simulink model "single_phase_inverter"  (R2026b)
settings: Solver=ode23tb  StopTime=simlength  FixedStep=tc  MaxStep=glb_time.tc
values from neighbouring files (symbols this model uses):
  afe_ctrl = param.afe.ctrl    [init_model.m]
  glb_time = param.glb_time    [init_model.m]
  grid_emu = param.grid.emu    [init_model.m]
  kepsilon = param.spinv.kepsilon    [init_model.m]
  omega_set = param.spinv.omega_set    [init_model.m]
  output_transformer = param.trafo_load.output_transformer    [init_model.m]
  single_phase_inverter_ctrl = param.spinv.ctrl    [init_model.m]
  time_step_ref_1 = param.spinv.ref.time_step_ref_1    [init_model.m]
  time_step_ref_2 = param.spinv.ref.time_step_ref_2    [init_model.m]
  time_step_ref_3 = param.spinv.ref.time_step_ref_3    [init_model.m]
undefined symbols (not defined in the file or in its folder): hwdata
libraries: fl_lib x49, nesl_utility x27, single_phase_transformer_lib x3, phase_shift_filter x2, phase_shift_filter_ccaller x2, lithium_ion_battery x1, three_phase_voltage_emulator x1, power_meter_iec x1, single_phase_transformer x1, three_phase_diode_rectifier x1, three_phase_diode_rectifier_with_thermal_model x1, full_bridge_mosfet_based_with_thermal_model x1
(part 1 of 4)
settings Model: Creator=LTNBDA  LastModifiedBy=d.bagnara
settings SolverCC: AutoInsertRateTranBlk=on  SolverResetMethod=Robust  ZeroCrossAlgorithm=Adaptive  ZeroCrossControl=DisableAll
settings DataIOCC: DSMLogging=off  LimitDataPoints=on  MaxDataPoints=1  ReturnWorkspaceOutputs=off  SaveFormat=Array  SaveOutput=off  SaveTime=off  SignalLogging=off  SignalLoggingSaveFormat=ModelDataLogs
settings OptimizationCC: EfficientMapNaN2IntZero=off  LifeSpan=inf  MemsetInitFltsAndDblsToZero=off
settings DebuggingCC: ArithmeticOperatorsInVariantConditions=warning  FcnCallInpInsideContextMsg=warning  IgnoredZcDiagnostic=none  MergeDetectMultiDrivingBlocksExec=none  MultiTaskCondExecSysMsg=none  MultiTaskDSMMsg=warning  MultiTaskRateTransMsg=warning  SFNoUnconditionalDefaultTransitionDiag=warning  SFUnexpectedBacktrackingDiag=warning  SaveWithParameterizedLinksMsg=none  SignalResolutionControl=TryResolveAllWithWarning  SolverPrmCheckMsg=warning  StateNameClashWarn=warning
settings HardwareCC: ProdEndianess=Unspecified  ProdEqTarget=off  ProdHWDeviceType=Generic->64-bit Embedded Processor (LP64)  ProdIntDivRoundTo=Undefined  ProdLargestAtomicFloat=None  TargetEndianess=LittleEndian  TargetHWDeviceType=MATLAB Host  TargetIntDivRoundTo=Zero  TargetLongLongMode=on
settings ModelReferenceCC: PropagateSignalLabelsOutOfModel=off
settings SFSimCC: CustomCodeUndefinedFunction=UseInterfaceOnly  SimUseLocalCustomCode=off
settings SFSimCC: SimCustomHeaderCode=|
  | #include "phase_shift_flt_simulink.h"
  | #include "sv_pwm.h"
  | #include "rpi.h"
  | #include "rpi_simulink.h"
  | #include "first_harmonic_tracker.h"
  | #include "dqvector_pi.h"
  | #include "dqvector_pi_simulink.h"
  | #include "sv_pwm_simulink.h"
  | #include "dqpll_grid.h"
  | #include "first_harmonic_tracker_simulink.h"
  | #include "dqpll_grid_simulink.h"
  | #include "phase_shift_flt.h"
  | #include "math_f.h"
  | #include "linear_double_integrator_observer_simulink.h"
  | #include "linear_double_integrator_observer.h"
  | #include "sogi_flt_simulink.h"
  | #include "sogi_flt.h"
settings SFSimCC: SimUserIncludeDirs=|
  | include
  | src
settings SFSimCC: SimUserSources=|
  | "rpi.c"
  | "rpi_simulink.c"
  | "dqvector_pi_simulink.c"
  | "dqvector_pi.c"
  | "sv_pwm_simulink.c"
  | "sv_pwm.c"
  | "first_harmonic_tracker_simulink.c"
  | "first_harmonic_tracker.c"
  | "dqpll_grid_simulink.c"
  | "dqpll_grid.c"
  | "phase_shift_flt_simulink.c"
  | "phase_shift_flt.c"
  | "linear_double_integrator_observer_simulink.c"
  | "linear_double_integrator_observer.c"
  | "sogi_flt_simulink.c"
  | "sogi_flt.c"
settings RTWCC: RTWUseLocalCustomCode=off
settings CodeAppCC: StateflowObjectComments=on
settings GRTTargetCC: CombineOutputUpdateFcns=off  GRTInterface=on  TargetLangStandard=C89/C90 (ANSI)
settings ConfigComp: CovExternalEMLEnable=off  CovSaveCumulativeToWorkspaceVar=on  CovSaveSingleToWorkspaceVar=on
settings SimscapeCC: SimscapeNormalizeSystem=off  SimscapeUseEnergyAccounting=off

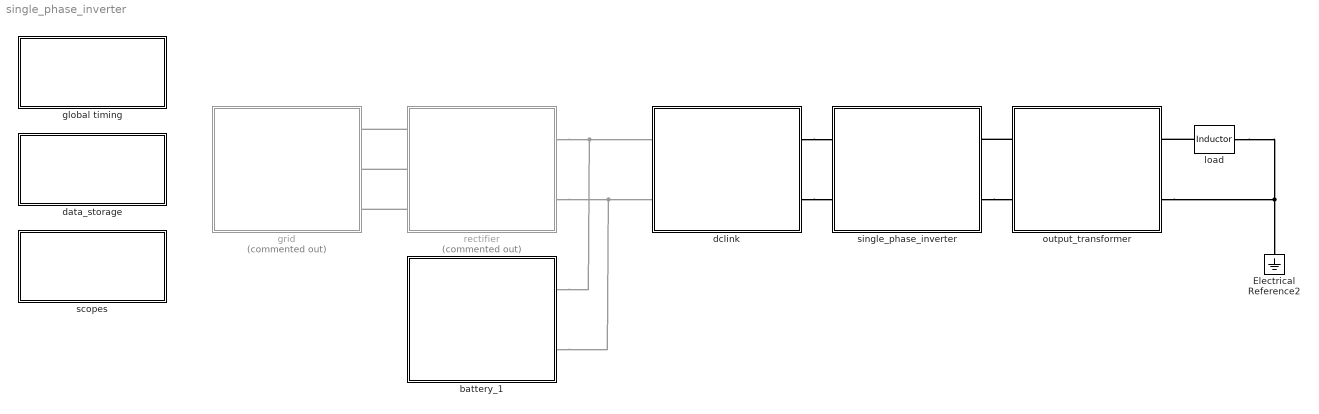
== system single_phase_inverter ==
  Electrical Reference2 : fl_lib/Electrical/Electrical Elements/Electrical Reference
  battery_1 : Subsystem
  data_storage : Subsystem
  dclink : Subsystem
  global timing : Subsystem
  grid : Subsystem  Commented=on
  load : fl_lib/Electrical/Electrical Elements/Inductor  l=lload H  r=rload Ohm  g=1e-9 1/Ohm  i_specify=off  i_priority=None  i=0 A  i_nominal_specify=off  i_nominal_value=1  i_nominal_unit=A  v_specify=off  v_priority=None  v=0 V  v_nominal_specify=off  v_nominal_value=1  v_nominal_unit=V  i_L_specify=off  i_L_priority=High  i_L=0 A  i_L_nominal_specify=off  i_L_nominal_value=1  i_L_nominal_unit=A
  output_transformer : Subsystem
  rectifier : Subsystem  Commented=on
  scopes : Subsystem
  single_phase_inverter : Subsystem
  connections:
  dclink/RConn2 -- single_phase_inverter/LConn2
  dclink/RConn1 -- single_phase_inverter/LConn1
  rectifier/RConn1 -- battery_1/RConn1 -- dclink/LConn1
  rectifier/RConn2 -- battery_1/RConn2 -- dclink/LConn2
  output_transformer/LConn1 -- single_phase_inverter/RConn1
  single_phase_inverter/RConn2 -- output_transformer/LConn2
  output_transformer/RConn2 -- load/RConn1 -- Electrical Reference2/LConn1
  load/LConn1 -- output_transformer/RConn1
  rectifier/LConn3 -- grid/RConn3
  rectifier/LConn2 -- grid/RConn2
  rectifier/LConn1 -- grid/RConn1

== system single_phase_inverter/battery_1 ==
  Electrical Reference : fl_lib/Electrical/Electrical Elements/Electrical Reference
  Inductor : fl_lib/Electrical/Electrical Elements/Inductor  l=1e-3 H  r=0 Ohm  g=1e-9 1/Ohm  i_specify=off  i_priority=None  i=0 A  i_nominal_specify=off  i_nominal_value=1  i_nominal_unit=A  v_specify=off  v_priority=None  v=0 V  v_nominal_specify=off  v_nominal_value=1  v_nominal_unit=V  i_L_specify=off  i_L_priority=High  i_L=0 A  i_L_nominal_specify=off  i_L_nominal_value=1  i_L_nominal_unit=A
  Solver Configuration : nesl_utility/Solver Configuration  PhysicalDomain=network_engine_domain  SubClassName=solver  LeftPortType=input  RightPortType=generic  Tones=[]  Harmonics=[]  SimulateNoise=off  Profile=off  UseLocalSampling=off  EnableSwitchedLinearOptims=on  FrequencyDomain=off  UseCCode=off  RelTol=0.001  AbsTol=0.001  MinStep=1e-09  ToWorkspace=off  RevertToSquareIcSolve=off  NumHomotopyIterations=100  PhasorMode=off  PhasorModeNumHarmonics=1  ConsistencySolver=NEWTON_FTOL  CanonicalOrdering=UNORDERED  OptimizeIntermediates=UNOPTIMIZED  MulticoreSolverChoice=BACKWARD_EULER  IndexReductionMethod=DerivativeReplacement  DoDC=on  ResidualTolerance=1e-3  ConsistencyTolSource=GLOBAL  ConsistencyAbsTol=0.001  ConsistencyRelTol=0.001  ConsistencyTolFactor=0.001  UseLocalSolver=on  LocalSolverChoice=NE_BACKWARD_EULER_ADVANCER  ResolveIndetEquations=on  FunctionEvalNumThread=1  LocalSolverSampleTime=glb_time.tc  DoFixedCost=on  MaxNonlinIter=nonlinear_iterations  MaxModeIter=2  ComputeImpulses=off  ImpulseIterations=2  LinearAlgebra=auto  LinearAlgebraNumThread=0  EquationFormulation=NE_TIME_EF  DelaysMemoryBudget=1024  AutomaticFiltering=on  FilteringTimeConstant=0.001  PartitionStorageMethod=AS_NEEDED  PartitionMemoryBudget=1024  PartitionMethod=BALANCED  MultibodyUseLocalSolver=off  MultibodyLocalSolverChoice=ODE1  MultibodyLocalSolverSampleTime=0.001
  To Workspace14 : ToWorkspace  VariableName=battery_1_data_sim  SampleTime=glb_time.tc
      settings: MaxDataPoints=glb_time.Nc  Decimation=glb_time.decimation_tc
  lithium ion battery : Scope
      settings: ActiveDisplayYMinimum=-808.27997881012811  ActiveDisplayYMaximum=1287.7546757937268  DataLoggingVariableName=ScopeData3
  lithium_ion_battery : lithium_ion_battery/lithium_ion_battery  Q=lithium_ion_battery_1.Q  number_of_cells=lithium_ion_battery_1.number_of_cells  E_1=lithium_ion_battery_1.E_1  E0=lithium_ion_battery_1.E0  E1=lithium_ion_battery_1.E1  E2=lithium_ion_battery_1.E2  E3=lithium_ion_battery_1.E3  Elog=lithium_ion_battery_1.Elog  R0=lithium_ion_battery_1.R0  R1=lithium_ion_battery_1.R1  C1=lithium_ion_battery_1.C1  M=lithium_ion_battery_1.M  alpha=lithium_ion_battery_1.alpha  soc_init=lithium_ion_battery_1.soc_init  ts_battery=glb_time.ts_dab  q1Kalman=lithium_ion_battery_1.q1Kalman  q2Kalman=lithium_ion_battery_1.q2Kalman  q3Kalman=lithium_ion_battery_1.q3Kalman  rKalman=lithium_ion_battery_1.rKalman  tc=glb_time.tc  enable_white_noise_m=0  battery_voltage_init_m=param.battery.nominal_battery_voltage_1
  single_phase_ui_measure : Subsystem
  dc(+) : PMIOPort  Side=Right
  dc(-) : PMIOPort  Port=2  Side=Right
  wires:
  lithium_ion_battery/1 -> To Workspace14/1, lithium ion battery/1
  connections:
  lithium_ion_battery/RConn2 -- single_phase_ui_measure/LConn2 -- Solver Configuration/RConn1 -- Electrical Reference/LConn1
  single_phase_ui_measure/RConn1 -- dc(+)/RConn1
  Inductor/LConn1 -- lithium_ion_battery/RConn1
  dc(-)/RConn1 -- single_phase_ui_measure/RConn2
  single_phase_ui_measure/LConn1 -- Inductor/RConn1

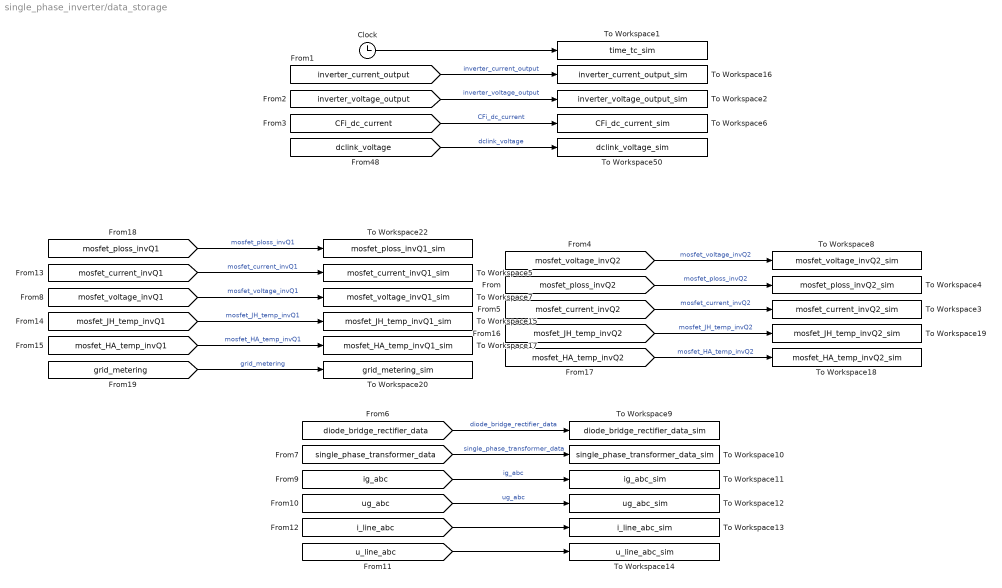
== system single_phase_inverter/data_storage ==
  Clock : Clock
  To Workspace1 : ToWorkspace  VariableName=time_tc_sim  SampleTime=glb_time.tc
      settings: MaxDataPoints=glb_time.Nc  Decimation=glb_time.decimation_tc
  To Workspace10 : ToWorkspace  VariableName=single_phase_transformer_data_sim  SampleTime=glb_time.tc
      settings: MaxDataPoints=glb_time.Nc  Decimation=glb_time.decimation_tc
  To Workspace11 : ToWorkspace  VariableName=ig_abc_sim  SampleTime=glb_time.tc
      settings: MaxDataPoints=glb_time.Nc  Decimation=glb_time.decimation_tc
  To Workspace12 : ToWorkspace  VariableName=ug_abc_sim  SampleTime=glb_time.tc
      settings: MaxDataPoints=glb_time.Nc  Decimation=glb_time.decimation_tc
  To Workspace13 : ToWorkspace  VariableName=i_line_abc_sim  SampleTime=glb_time.tc
      settings: MaxDataPoints=glb_time.Nc  Decimation=glb_time.decimation_tc
  To Workspace14 : ToWorkspace  VariableName=u_line_abc_sim  SampleTime=glb_time.tc
      settings: MaxDataPoints=glb_time.Nc  Decimation=glb_time.decimation_tc
  To Workspace15 : ToWorkspace  VariableName=mosfet_JH_temp_invQ1_sim  SampleTime=glb_time.tc
      settings: MaxDataPoints=glb_time.Nc  Decimation=glb_time.decimation_tc
  To Workspace16 : ToWorkspace  VariableName=inverter_current_output_sim  SampleTime=glb_time.tc
      settings: MaxDataPoints=glb_time.Nc  Decimation=glb_time.decimation_tc
  To Workspace17 : ToWorkspace  VariableName=mosfet_HA_temp_invQ1_sim  SampleTime=glb_time.tc
      settings: MaxDataPoints=glb_time.Nc  Decimation=glb_time.decimation_tc
  To Workspace18 : ToWorkspace  VariableName=mosfet_HA_temp_invQ2_sim  SampleTime=glb_time.tc
      settings: MaxDataPoints=glb_time.Nc  Decimation=glb_time.decimation_tc
  To Workspace19 : ToWorkspace  VariableName=mosfet_JH_temp_invQ2_sim  SampleTime=glb_time.tc
      settings: MaxDataPoints=glb_time.Nc  Decimation=glb_time.decimation_tc
  To Workspace2 : ToWorkspace  VariableName=inverter_voltage_output_sim  SampleTime=glb_time.tc
      settings: MaxDataPoints=glb_time.Nc  Decimation=glb_time.decimation_tc
  To Workspace20 : ToWorkspace  VariableName=grid_metering_sim  SampleTime=glb_time.tc
      settings: MaxDataPoints=glb_time.Nc  Decimation=glb_time.decimation_tc
  To Workspace22 : ToWorkspace  VariableName=mosfet_ploss_invQ1_sim  SampleTime=glb_time.tc
      settings: MaxDataPoints=glb_time.Nc  Decimation=glb_time.decimation_tc
  To Workspace3 : ToWorkspace  VariableName=mosfet_current_invQ2_sim  SampleTime=glb_time.tc
      settings: MaxDataPoints=glb_time.Nc  Decimation=glb_time.decimation_tc
  To Workspace4 : ToWorkspace  VariableName=mosfet_ploss_invQ2_sim  SampleTime=glb_time.tc
      settings: MaxDataPoints=glb_time.Nc  Decimation=glb_time.decimation_tc
  To Workspace5 : ToWorkspace  VariableName=mosfet_current_invQ1_sim  SampleTime=glb_time.tc
      settings: MaxDataPoints=glb_time.Nc  Decimation=glb_time.decimation_tc
  To Workspace50 : ToWorkspace  VariableName=dclink_voltage_sim  SampleTime=glb_time.tc
      settings: MaxDataPoints=glb_time.Nc  Decimation=glb_time.decimation_tc
  To Workspace6 : ToWorkspace  VariableName=CFi_dc_current_sim  SampleTime=glb_time.tc
      settings: MaxDataPoints=glb_time.Nc  Decimation=glb_time.decimation_tc
  To Workspace7 : ToWorkspace  VariableName=mosfet_voltage_invQ1_sim  SampleTime=glb_time.tc
      settings: MaxDataPoints=glb_time.Nc  Decimation=glb_time.decimation_tc
  To Workspace8 : ToWorkspace  VariableName=mosfet_voltage_invQ2_sim  SampleTime=glb_time.tc
      settings: MaxDataPoints=glb_time.Nc  Decimation=glb_time.decimation_tc
  To Workspace9 : ToWorkspace  VariableName=diode_bridge_rectifier_data_sim  SampleTime=glb_time.tc
      settings: MaxDataPoints=glb_time.Nc  Decimation=glb_time.decimation_tc
  wires:
  Clock/1 -> To Workspace1/1
  [inverter_current_output] -> To Workspace16/1  "inverter_current_output"
  [inverter_voltage_output] -> To Workspace2/1  "inverter_voltage_output"
  [CFi_dc_current] -> To Workspace6/1  "CFi_dc_current"
  [mosfet_ploss_invQ1] -> To Workspace22/1  "mosfet_ploss_invQ1"
  [dclink_voltage] -> To Workspace50/1  "dclink_voltage"
  [mosfet_current_invQ1] -> To Workspace5/1  "mosfet_current_invQ1"
  [mosfet_current_invQ2] -> To Workspace3/1  "mosfet_current_invQ2"
  [mosfet_ploss_invQ2] -> To Workspace4/1  "mosfet_ploss_invQ2"
  [mosfet_voltage_invQ1] -> To Workspace7/1  "mosfet_voltage_invQ1"
  [mosfet_voltage_invQ2] -> To Workspace8/1  "mosfet_voltage_invQ2"
  [diode_bridge_rectifier_data] -> To Workspace9/1  "diode_bridge_rectifier_data"
  [single_phase_transformer_data] -> To Workspace10/1  "single_phase_transformer_data"
  [ig_abc] -> To Workspace11/1  "ig_abc"
  [ug_abc] -> To Workspace12/1  "ug_abc"
  [i_line_abc] -> To Workspace13/1
  [u_line_abc] -> To Workspace14/1
  [mosfet_JH_temp_invQ1] -> To Workspace15/1  "mosfet_JH_temp_invQ1"
  [mosfet_HA_temp_invQ1] -> To Workspace17/1  "mosfet_HA_temp_invQ1"
  [mosfet_JH_temp_invQ2] -> To Workspace19/1  "mosfet_JH_temp_invQ2"
  [mosfet_HA_temp_invQ2] -> To Workspace18/1  "mosfet_HA_temp_invQ2"
  [grid_metering] -> To Workspace20/1  "grid_metering"

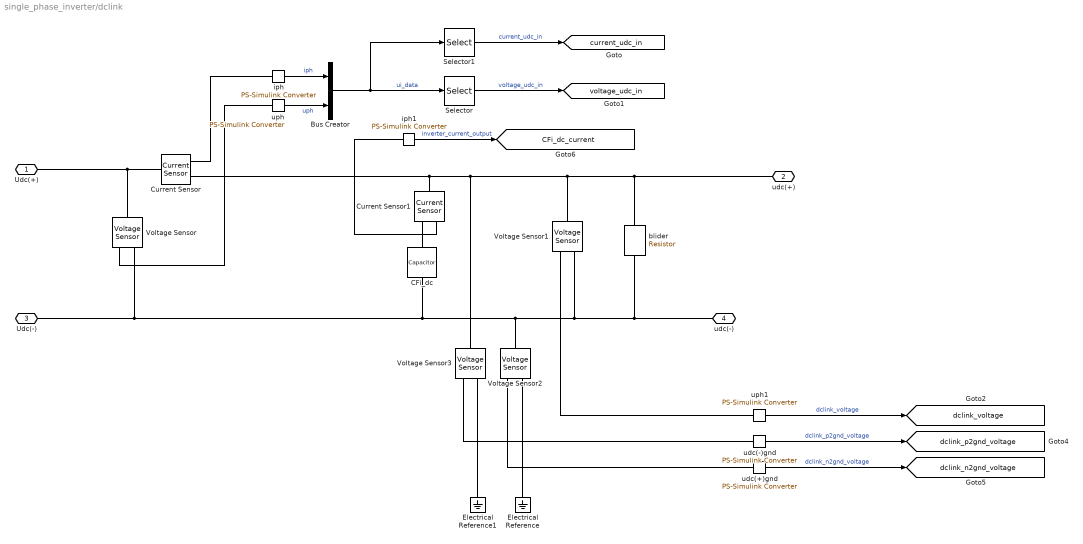
== system single_phase_inverter/dclink ==
  Bus Creator : BusCreator  Inputs=2
  CFi_dc : fl_lib/Electrical/Electrical Elements/Capacitor  c=hwdata.single_phase_inverter.CFi F  r=hwdata.single_phase_inverter.RCFi Ohm  g=0 1/Ohm  i_specify=off  i_priority=None  i=0 A  i_nominal_specify=off  i_nominal_value=1  i_nominal_unit=A  v_specify=off  v_priority=None  v=0 V  v_nominal_specify=off  v_nominal_value=1  v_nominal_unit=V  vc_specify=off  vc_priority=High  vc=0 V  vc_nominal_specify=off  vc_nominal_value=1  vc_nominal_unit=V
  Current Sensor : fl_lib/Electrical/Electrical Sensors/Current Sensor
  Current Sensor1 : fl_lib/Electrical/Electrical Sensors/Current Sensor
  Electrical Reference : fl_lib/Electrical/Electrical Elements/Electrical Reference
  Electrical Reference1 : fl_lib/Electrical/Electrical Elements/Electrical Reference
  Selector : Selector  InputPortWidth=2  IndexOptions=Index vector (dialog)  Indices=2  OutputSizes=1  RuntimeRangeChecks=off
  Selector1 : Selector  InputPortWidth=2  IndexOptions=Index vector (dialog)  Indices=1  OutputSizes=1  RuntimeRangeChecks=off
  Voltage Sensor{,1..3} (4 alike) : fl_lib/Electrical/Electrical Sensors/Voltage Sensor
  blider : fl_lib/Electrical/Electrical Elements/Resistor  R=1200 Ohm  i_specify=off  i_priority=None  i=0 A  i_nominal_specify=off  i_nominal_value=1  i_nominal_unit=A  v_specify=off  v_priority=None  v=0 V  v_nominal_specify=off  v_nominal_value=1  v_nominal_unit=V
  iph : nesl_utility/PS-Simulink Converter  PhysicalDomain=network_engine_domain  SubClassName=ps_output  LeftPortType=input  RightPortType=output  PseudoPeriodic=off  Frequencies=[]  VectorFormat=1-D array  Unit=A  AffineConversion=off
  iph1 : nesl_utility/PS-Simulink Converter  PhysicalDomain=network_engine_domain  SubClassName=ps_output  LeftPortType=input  RightPortType=output  PseudoPeriodic=off  Frequencies=[]  VectorFormat=1-D array  Unit=A  AffineConversion=off
  udc(+)gnd : nesl_utility/PS-Simulink Converter  PhysicalDomain=network_engine_domain  SubClassName=ps_output  LeftPortType=input  RightPortType=output  PseudoPeriodic=off  Frequencies=[]  VectorFormat=1-D array  Unit=V  AffineConversion=off
  udc(-)gnd : nesl_utility/PS-Simulink Converter  PhysicalDomain=network_engine_domain  SubClassName=ps_output  LeftPortType=input  RightPortType=output  PseudoPeriodic=off  Frequencies=[]  VectorFormat=1-D array  Unit=V  AffineConversion=off
  uph : nesl_utility/PS-Simulink Converter  PhysicalDomain=network_engine_domain  SubClassName=ps_output  LeftPortType=input  RightPortType=output  PseudoPeriodic=off  Frequencies=[]  VectorFormat=1-D array  Unit=V  AffineConversion=off
  uph1 : nesl_utility/PS-Simulink Converter  PhysicalDomain=network_engine_domain  SubClassName=ps_output  LeftPortType=input  RightPortType=output  PseudoPeriodic=off  Frequencies=[]  VectorFormat=1-D array  Unit=V  AffineConversion=off
  Udc(+) : PMIOPort  Side=Left
  udc(+) : PMIOPort  Port=2  Side=Right
  Udc(-) : PMIOPort  Port=3  Side=Left
  udc(-) : PMIOPort  Port=4  Side=Right
  tag scope: CFi_dc_current=global, current_udc_in=global, dclink_n2gnd_voltage=global, dclink_p2gnd_voltage=global, dclink_voltage=global, voltage_udc_in=global
  wires:
  Bus Creator/1 -> Selector/1, Selector1/1  "ui_data"
  iph/1 -> Bus Creator/1  "iph"
  uph/1 -> Bus Creator/2  "uph"
  Selector1/1 -> [current_udc_in]  "current_udc_in"
  Selector/1 -> [voltage_udc_in]  "voltage_udc_in"
  iph1/1 -> [CFi_dc_current]  "inverter_current_output"
  udc(+)gnd/1 -> [dclink_n2gnd_voltage]  "dclink_n2gnd_voltage"
  uph1/1 -> [dclink_voltage]  "dclink_voltage"
  udc(-)gnd/1 -> [dclink_p2gnd_voltage]  "dclink_p2gnd_voltage"
  connections:
  iph/LConn1 -- Current Sensor/RConn1
  Voltage Sensor/LConn1 -- Current Sensor/LConn1 -- Udc(+)/RConn1
  Voltage Sensor/RConn1 -- uph/LConn1
  CFi_dc/RConn1 -- Voltage Sensor1/RConn2 -- udc(-)/RConn1 -- blider/RConn1 -- Voltage Sensor2/LConn1 -- Voltage Sensor/RConn2 -- Udc(-)/RConn1
  udc(+)/RConn1 -- blider/LConn1 -- Voltage Sensor1/LConn1 -- Voltage Sensor3/LConn1 -- Current Sensor/RConn2 -- Current Sensor1/LConn1
  Current Sensor1/RConn2 -- CFi_dc/LConn1
  Electrical Reference1/LConn1 -- Voltage Sensor3/RConn2
  udc(-)gnd/LConn1 -- Voltage Sensor3/RConn1
  Voltage Sensor2/RConn1 -- udc(+)gnd/LConn1
  Electrical Reference/LConn1 -- Voltage Sensor2/RConn2
  Voltage Sensor1/RConn1 -- uph1/LConn1
  Current Sensor1/RConn1 -- iph1/LConn1

== system single_phase_inverter/global timing ==
  Unit Delay : UnitDelay  SampleTime=glb_time.tc
  time_afe1 : Subsystem  mask{k=1}
      mask prompts: k "Time Gain"
      mask Display:
      | disp('time-gen');
      | port_label('input', 1, 'crt');
      | port_label('output', 1, 'tout');
  time_afe3 : Subsystem  mask{k=1}
      mask prompts: k "Time Gain"
      mask Display:
      | disp('time-gen');
      | port_label('output', 1, 'tout');
  tag scope: master_time=global, time_inv_module_1=global
  wires:
  time_afe1/1(Out1) -> [time_inv_module_1]
  time_afe3/1(Out1) -> [master_time]
  [local_time_corr_llc_mod1] -> Unit Delay/1
  Unit Delay/1 -> time_afe1/1(correction_time)

== system single_phase_inverter/grid ==
  grid_emulator : Subsystem
  power meter iec : power_meter_iec/power meter iec  period=10e-3  ts=glb_time.tc  enable_time=0.025
  threephase_vi_measures : Subsystem
  ua : PMIOPort  Side=Right
  ub : PMIOPort  Port=2  Side=Right
  uc : PMIOPort  Port=3  Side=Right
  tag scope: grid_metering=global
  wires:
  [ug_abc] -> power meter iec/2
  [grid_pulsation_emulator] -> power meter iec/4
  [ig_abc] -> power meter iec/3
  [grid_phase_emulator] -> power meter iec/1
  power meter iec/1 -> [grid_metering]
  connections:
  threephase_vi_measures/LConn3 -- grid_emulator/RConn3
  threephase_vi_measures/LConn1 -- grid_emulator/RConn1
  threephase_vi_measures/RConn2 -- ub/RConn1
  threephase_vi_measures/LConn2 -- grid_emulator/RConn2
  threephase_vi_measures/RConn1 -- ua/RConn1
  threephase_vi_measures/RConn3 -- uc/RConn1

== system single_phase_inverter/output_transformer ==
  single_phase_transformer : single_phase_transformer/single_phase_transformer  lm_trafo=output_transformer.Lm1  m1=output_transformer.n1  m2=output_transformer.n2  rd1_trafo=output_transformer.Rd1  rd2_trafo=0  ld1_trafo=2*output_transformer.Ld1  ld2_trafo=0  rfe_trafo=output_transformer.Rfe1  length_core=1  mu0=1.256637e-6  mur=1200
  single_phase_transformer - scope : Scope
      settings: ActiveDisplayYMinimum=-52667.127888169394  ActiveDisplayYMaximum=52594.361496045676  DataLoggingVariableName=ScopeData11
  u1(+) : PMIOPort  Side=Left
  u2(+) : PMIOPort  Port=2  Side=Right
  u1(-) : PMIOPort  Port=3  Side=Left
  u2(-) : PMIOPort  Port=4  Side=Right
  tag scope: single_phase_transformer_data=global
  wires:
  single_phase_transformer/1 -> [single_phase_transformer_data], single_phase_transformer - scope/1
  connections:
  single_phase_transformer/LConn2 -- u1(-)/RConn1
  single_phase_transformer/LConn1 -- u1(+)/RConn1
  single_phase_transformer/RConn1 -- u2(+)/RConn1
  single_phase_transformer/RConn2 -- u2(-)/RConn1

== system single_phase_inverter/rectifier ==
  H5_filter : Subsystem  Commented=on
  H7_filter : Subsystem  Commented=on
  three phase diode rectifier : three_phase_diode_rectifier/three phase diode rectifier  Commented=on  Vf_diode_rectifier=diode.rectifier.Vf  Rdon_diode_rectifier=diode.rectifier.Rdon  Csnubber=igbt.inv.Csnubber  Rsnubber=igbt.inv.Rsnubber
  three_phase_diode_rectifier_with_thermal_model : three_phase_diode_rectifier_with_thermal_model/three_phase_diode_rectifier_with_thermal_model  Vf_diode_rectifier=diode.rectifier.Vf  Rdon_diode_rectifier=diode.rectifier.Rdon  mass_heatsink_m=heatsink.no_weight  specific_heat_m=heatsink.cp  rth_diode_JH_m=igbt.inv.Rth_diode_JH  rth_diode_HA_m=Rth_mosfet_HA  Csnubber=igbt.inv.Csnubber  Rsnubber=igbt.inv.Rsnubber
      link override diode_3/Goto2: GotoTag=diode3_JH_temperature
  us_a : PMIOPort  Side=Left
  us_b : PMIOPort  Port=2  Side=Left
  us_c : PMIOPort  Port=3  Side=Left
  Udc(+) : PMIOPort  Port=4  Side=Right
  Udc(-) : PMIOPort  Port=5  Side=Right
  tag scope: diode_bridge_rectifier_data=global
  wires:
  three_phase_diode_rectifier_with_thermal_model/1 -> [diode_bridge_rectifier_data]
  connections:
  Udc(+)/RConn1 -- three_phase_diode_rectifier_with_thermal_model/RConn1 -- three phase diode rectifier/RConn1
  Udc(-)/RConn1 -- three_phase_diode_rectifier_with_thermal_model/RConn2 -- three phase diode rectifier/RConn2
  H5_filter/LConn1 -- us_a/RConn1 -- three_phase_diode_rectifier_with_thermal_model/LConn1 -- three phase diode rectifier/LConn1 -- H7_filter/LConn1
  H5_filter/LConn2 -- us_b/RConn1 -- three phase diode rectifier/LConn2 -- three_phase_diode_rectifier_with_thermal_model/LConn2 -- H7_filter/LConn2
  H5_filter/LConn3 -- us_c/RConn1 -- three_phase_diode_rectifier_with_thermal_model/LConn3 -- three phase diode rectifier/LConn3 -- H7_filter/LConn3

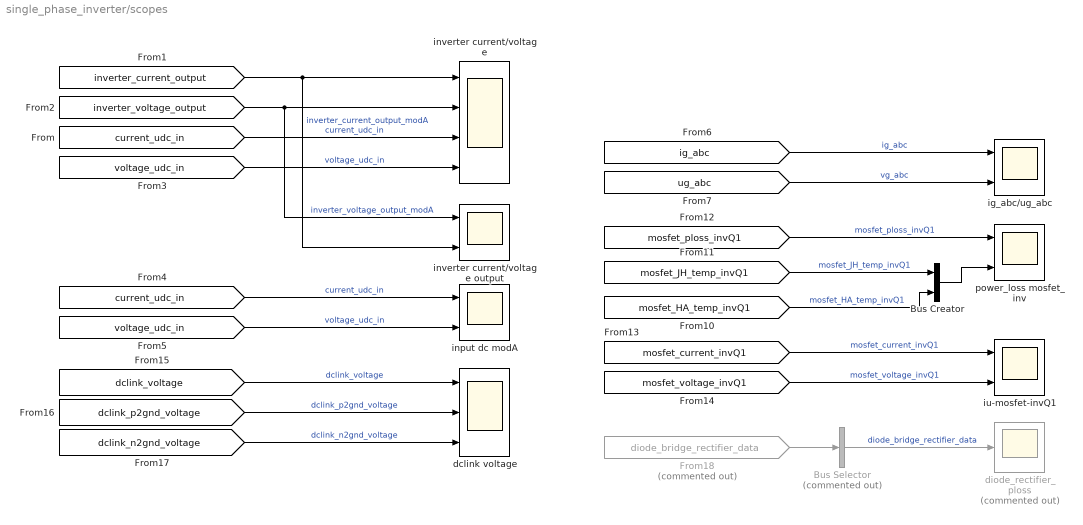
== system single_phase_inverter/scopes ==
  Bus Creator : BusCreator  Inputs=2
  Bus Selector : BusSelector  Commented=on  OutputSignals=diode1_ploss,diode6_ploss,diode5_ploss,diode4_ploss,diode3_ploss,diode2_ploss  OutputAsBus=on
  From18 : From  Commented=on  GotoTag=diode_bridge_rectifier_data
  dclink voltage : Scope  NumInputPorts=3
      settings: SampleTime=glb_time.tc  ActiveDisplayString=3  ActiveDisplayYMinimum=-458.99159991109462  ActiveDisplayYMaximum=51.251012962530893  DataLoggingVariableName=ScopeData9
  diode_rectifier_ploss : Scope  Commented=on
      settings: ActiveDisplayYMinimum=-388.41488046396341  ActiveDisplayYMaximum=3494.091610714474  DataLoggingVariableName=ScopeData13
  ig_abc/ug_abc : Scope  NumInputPorts=2
      settings: SampleTime=glb_time.tc  ActiveDisplayYMinimum=-432.03154642527051  ActiveDisplayYMaximum=443.5760585618213  DataLoggingVariableName=ScopeData5
  input dc modA : Scope  NumInputPorts=2
      settings: SampleTime=glb_time.tc  ActiveDisplayYMinimum=-178.52925477225054  ActiveDisplayYMaximum=1606.7629734926184  DataLoggingVariableName=ScopeData4
  inverter current/voltage : Scope  NumInputPorts=4
      settings: ActiveDisplayString=3  ActiveDisplayYMinimum=-178.52926094214885  ActiveDisplayYMaximum=1606.7629741781627
  inverter current/voltage output : Scope  NumInputPorts=2
      settings: ActiveDisplayYMinimum=-156.50578790248869  ActiveDisplayYMaximum=540.48726644352541
  iu-mosfet-invQ1 : Scope  NumInputPorts=2
      settings: SampleTime=glb_time.tc  ActiveDisplayYMinimum=-1884.5917198054758  ActiveDisplayYMaximum=2532.7760155502147  DataLoggingVariableName=ScopeData7
  power_loss mosfet_inv : Scope  NumInputPorts=2
      settings: SampleTime=glb_time.tc  ActiveDisplayYMinimum=-70.3597503046535  ActiveDisplayYMaximum=633.23512274412  DataLoggingVariableName=ScopeData6
  wires:
  [current_udc_in] -> inverter current/voltage/3  "current_udc_in"
  [inverter_voltage_output] -> inverter current/voltage/2, inverter current/voltage output/1  "inverter_voltage_output_modA"
  [inverter_current_output] -> inverter current/voltage/1, inverter current/voltage output/2  "inverter_current_output_modA"
  [voltage_udc_in] -> inverter current/voltage/4  "voltage_udc_in"
  [current_udc_in] -> input dc modA/1  "current_udc_in"
  [voltage_udc_in] -> input dc modA/2  "voltage_udc_in"
  [ug_abc] -> ig_abc/ug_abc/2  "vg_abc"
  [ig_abc] -> ig_abc/ug_abc/1  "ig_abc"
  [mosfet_ploss_invQ1] -> power_loss mosfet_inv/1  "mosfet_ploss_invQ1"
  [mosfet_JH_temp_invQ1] -> Bus Creator/1  "mosfet_JH_temp_invQ1"
  [mosfet_HA_temp_invQ1] -> Bus Creator/2  "mosfet_HA_temp_invQ1"
  Bus Creator/1 -> power_loss mosfet_inv/2
  [mosfet_current_invQ1] -> iu-mosfet-invQ1/1  "mosfet_current_invQ1"
  [mosfet_voltage_invQ1] -> iu-mosfet-invQ1/2  "mosfet_voltage_invQ1"
  [dclink_voltage] -> dclink voltage/1  "dclink_voltage"
  [dclink_p2gnd_voltage] -> dclink voltage/2  "dclink_p2gnd_voltage"
  [dclink_n2gnd_voltage] -> dclink voltage/3  "dclink_n2gnd_voltage"
  From18/1 -> Bus Selector/1
  Bus Selector/1 -> diode_rectifier_ploss/1  "diode_bridge_rectifier_data"

== system single_phase_inverter/single_phase_inverter ==
  Current Sensor : fl_lib/Electrical/Electrical Sensors/Current Sensor
  Voltage Sensor1 : fl_lib/Electrical/Electrical Sensors/Voltage Sensor
  iph : nesl_utility/PS-Simulink Converter  PhysicalDomain=network_engine_domain  SubClassName=ps_output  LeftPortType=input  RightPortType=output  PseudoPeriodic=off  Frequencies=[]  VectorFormat=1-D array  Unit=A  AffineConversion=off
  single phase inverter : Subsystem
      settings: PortSchema="{\"entries\":[{\"content\":{\"sides\":[{\"content\":{\"connectorIds\":[\"LConn1\",\"LConn2\"]},\"type\":\"ConnectorPlacement.EquallySpacedRectSide\",\"uuid\":\"4fcf4fea-d38f-431b-8a91-be3ce9782faf\"},{\"content\":{\"connectorIds\":[\"RConn1\",\"RConn2\"],\"side\":\"RIGHT\"},\"type\":\"ConnectorPlacement.EquallySpacedRectSide\",\"uuid\":\"0aa56277-92e9-4e3b-84c7-43398254a4d8\"},{\"content\":{\"connectorIds\":[\"In1\"],\"side\":\"TOP\"},\"type\":\"ConnectorPlacement.EquallySpacedRectSide\",\"uuid\":\"5cd150dc-bcaf-4cd7-b2a8-3db203726730\"}]},\"type\":\"ConnectorPlacement.EquallySpacedConnector\",\"uuid\":\"bf8194c4-c327-4d40-bea4-f1e7617f80b4\"}],\"packageUris\":[\"http://schema.mathworks.com/mf0/Connector/R2020b\"],\"version\":\"1.0\"}"
  single phase inverter control : Subsystem
  uph1 : nesl_utility/PS-Simulink Converter  PhysicalDomain=network_engine_domain  SubClassName=ps_output  LeftPortType=input  RightPortType=output  PseudoPeriodic=off  Frequencies=[]  VectorFormat=1-D array  Unit=V  AffineConversion=off
  uac(+) : PMIOPort  Side=Right
  uac(-) : PMIOPort  Port=2  Side=Right
  udc(+) : PMIOPort  Port=3  Side=Left
  udc(-) : PMIOPort  Port=4  Side=Left
  tag scope: inverter_current_output=global, inverter_voltage_output=global
  wires:
  single phase inverter control/1(gate_cmds) -> single phase inverter/1(gate_commands)
  iph/1 -> [inverter_current_output]  "inverter_current_output"
  uph1/1 -> [inverter_voltage_output]  "inverter_voltage_output"
  connections:
  Current Sensor/LConn1 -- single phase inverter/LConn1
  uac(-)/RConn1 -- single phase inverter/LConn2 -- Voltage Sensor1/RConn2
  Voltage Sensor1/RConn1 -- uph1/LConn1
  iph/LConn1 -- Current Sensor/RConn1
  uac(+)/RConn1 -- Current Sensor/RConn2 -- Voltage Sensor1/LConn1
  udc(+)/RConn1 -- single phase inverter/RConn1
  udc(-)/RConn1 -- single phase inverter/RConn2

== system single_phase_inverter/battery_1/single_phase_ui_measure ==
  Bus Creator : BusCreator  Inputs=2
  Current Sensor : fl_lib/Electrical/Electrical Sensors/Current Sensor
  Selector : Selector  InputPortWidth=2  IndexOptions=Index vector (dialog)  Indices=2  OutputSizes=1  RuntimeRangeChecks=off
  Selector1 : Selector  InputPortWidth=2  IndexOptions=Index vector (dialog)  Indices=1  OutputSizes=1  RuntimeRangeChecks=off
  Terminator : Terminator
  Terminator1 : Terminator
  Voltage Sensor : fl_lib/Electrical/Electrical Sensors/Voltage Sensor
  dab input modA : Scope  NumInputPorts=2
      settings: SampleTime=glb_time.tc  ActiveDisplayYMinimum=1239.6508899029441  ActiveDisplayYMaximum=1249.6536701415532  DataLoggingVariableName=ScopeData2
  iph : nesl_utility/PS-Simulink Converter  PhysicalDomain=network_engine_domain  SubClassName=ps_output  LeftPortType=input  RightPortType=output  PseudoPeriodic=off  Frequencies=[]  VectorFormat=1-D array  Unit=A  AffineConversion=off
  uph : nesl_utility/PS-Simulink Converter  PhysicalDomain=network_engine_domain  SubClassName=ps_output  LeftPortType=input  RightPortType=output  PseudoPeriodic=off  Frequencies=[]  VectorFormat=1-D array  Unit=V  AffineConversion=off
  Udc(+) : PMIOPort  Side=Left
  udc(+) : PMIOPort  Port=2  Side=Right
  Udc(-) : PMIOPort  Port=3  Side=Left
  udc(-) : PMIOPort  Port=4  Side=Right
  tag scope: current_battery_1=global, voltage_battery_1=global
  wires:
  Bus Creator/1 -> Selector/1, Selector1/1  "ui_data"
  iph/1 -> Bus Creator/1  "iph"
  uph/1 -> Bus Creator/2  "uph"
  Selector1/1 -> [current_battery_1], dab input modA/1  "current_battery"
  Selector/1 -> dab input modA/2, [voltage_battery_1]  "voltage_battery"
  [current_battery_1] -> Terminator/1
  [voltage_battery_1] -> Terminator1/1
  connections:
  iph/LConn1 -- Current Sensor/RConn1
  Voltage Sensor/LConn1 -- Current Sensor/LConn1 -- Udc(+)/RConn1
  Current Sensor/RConn2 -- udc(+)/RConn1
  Voltage Sensor/RConn1 -- uph/LConn1
  Voltage Sensor/RConn2 -- Udc(-)/RConn1 -- udc(-)/RConn1

== system single_phase_inverter/global timing/time_afe1 ==
  correction_time : Inport
  Constant : Constant
  Gain : Gain  Gain=k
  Product : Product
  Sum : Sum  Inputs=|++
  time_1 : Clock
  Out1 : Outport
  wires:
  time_1/1 -> Gain/1
  Gain/1 -> Product/1
  Product/1 -> Out1/1
  correction_time/1 -> Sum/1
  Sum/1 -> Product/2
  Constant/1 -> Sum/2

== system single_phase_inverter/global timing/time_afe3 ==
  Gain : Gain  Gain=k
  time_1 : Clock
  Out1 : Outport
  wires:
  Gain/1 -> Out1/1
  time_1/1 -> Gain/1

== system single_phase_inverter/grid/grid_emulator ==
  3ph_Dyg : Subsystem
  Bus Selector : BusSelector  OutputSignals=ua_grid_emu,ub_grid_emu,uc_grid_emu
  Bus Selector1 : BusSelector  OutputSignals=gamma_grid_emulator,omega_grid_emulator
  Controlled Voltage Source : fl_lib/Electrical/Electrical Sources/Controlled Voltage Source
  Controlled Voltage Source1 : fl_lib/Electrical/Electrical Sources/Controlled Voltage Source
  Controlled Voltage Source2 : fl_lib/Electrical/Electrical Sources/Controlled Voltage Source
  Electrical Reference : fl_lib/Electrical/Electrical Elements/Electrical Reference
  Simulink-PS Converter : nesl_utility/Simulink-PS Converter  PhysicalDomain=network_engine_domain  SubClassName=ps_input  LeftPortType=input  RightPortType=output  PseudoPeriodic=off  Frequencies=[]  NoiseDistribution=none  NoiseParameters=[]  Unit=V  AffineConversion=on  FilteringAndDerivatives=provide  SimscapeFilterOrder=1  InputFilterTimeConstant=0.001  UdotUserProvided=0
  Simulink-PS Converter1 : nesl_utility/Simulink-PS Converter  PhysicalDomain=network_engine_domain  SubClassName=ps_input  LeftPortType=input  RightPortType=output  PseudoPeriodic=off  Frequencies=[]  NoiseDistribution=none  NoiseParameters=[]  Unit=V  AffineConversion=on  FilteringAndDerivatives=provide  SimscapeFilterOrder=1  InputFilterTimeConstant=0.001  UdotUserProvided=0
  Simulink-PS Converter2 : nesl_utility/Simulink-PS Converter  PhysicalDomain=network_engine_domain  SubClassName=ps_input  LeftPortType=input  RightPortType=output  PseudoPeriodic=off  Frequencies=[]  NoiseDistribution=none  NoiseParameters=[]  Unit=V  AffineConversion=on  FilteringAndDerivatives=provide  SimscapeFilterOrder=1  InputFilterTimeConstant=0.001  UdotUserProvided=0
  Solver Configuration : nesl_utility/Solver Configuration  PhysicalDomain=network_engine_domain  SubClassName=solver  LeftPortType=input  RightPortType=generic  Tones=[]  Harmonics=[]  SimulateNoise=off  Profile=off  UseLocalSampling=off  EnableSwitchedLinearOptims=on  FrequencyDomain=off  UseCCode=off  RelTol=0.001  AbsTol=0.001  MinStep=1e-09  ToWorkspace=off  RevertToSquareIcSolve=off  NumHomotopyIterations=100  PhasorMode=off  PhasorModeNumHarmonics=1  ConsistencySolver=NEWTON_XTOL_AFTER_FTOL  CanonicalOrdering=UNORDERED  OptimizeIntermediates=UNOPTIMIZED  MulticoreSolverChoice=BACKWARD_EULER  IndexReductionMethod=DerivativeReplacement  DoDC=on  ResidualTolerance=1e-09  ConsistencyTolSource=GLOBAL  ConsistencyAbsTol=0.001  ConsistencyRelTol=0.001  ConsistencyTolFactor=0.001  UseLocalSolver=on  LocalSolverChoice=NE_BACKWARD_EULER_ADVANCER  ResolveIndetEquations=on  FunctionEvalNumThread=1  LocalSolverSampleTime=glb_time.tc  DoFixedCost=on  MaxNonlinIter=3  MaxModeIter=2  ComputeImpulses=off  ImpulseIterations=2  LinearAlgebra=auto  LinearAlgebraNumThread=0  EquationFormulation=NE_TIME_EF  DelaysMemoryBudget=1024  AutomaticFiltering=on  FilteringTimeConstant=0.001  PartitionStorageMethod=AS_NEEDED  PartitionMemoryBudget=1024  PartitionMethod=BALANCED  MultibodyUseLocalSolver=off  MultibodyLocalSolverChoice=ODE1  MultibodyLocalSolverSampleTime=0.001
  three_phase_voltage_source_emulator : three_phase_voltage_emulator/three_phase_voltage_source_emulator  freq=50  ugrid_nom=400  vp_xi_pu=1  vp_eta_pu=0  vn_xi_pu=0  vn_eta_pu=0  fcut_lvrt=50
  threephase_vi_measures : Subsystem
  u1 : PMIOPort  Side=Right
  u2 : PMIOPort  Port=2  Side=Right
  u3 : PMIOPort  Port=3  Side=Right
  tag scope: grid_phase_emulator=global, grid_pulsation_emulator=global
  wires:
  Bus Selector/2 -> Simulink-PS Converter1/1  "<ub_grid_emu>"
  Bus Selector/3 -> Simulink-PS Converter2/1  "<uc_grid_emu>"
  Bus Selector/1 -> Simulink-PS Converter/1  "<ua_grid_emu>"
  three_phase_voltage_source_emulator/1 -> Bus Selector1/1, Bus Selector/1
  Bus Selector1/1 -> [grid_phase_emulator]  "<gamma_grid_emulator>"
  Bus Selector1/2 -> [grid_pulsation_emulator]  "<omega_grid_emulator>"
  connections:
  Simulink-PS Converter/RConn1 -- Controlled Voltage Source/RConn1
  Simulink-PS Converter1/RConn1 -- Controlled Voltage Source1/RConn1
  Simulink-PS Converter2/RConn1 -- Controlled Voltage Source2/RConn1
  Electrical Reference/LConn1 -- Solver Configuration/RConn1 -- Controlled Voltage Source/RConn2 -- Controlled Voltage Source1/RConn2 -- Controlled Voltage Source2/RConn2
  Controlled Voltage Source/LConn1 -- threephase_vi_measures/LConn1
  Controlled Voltage Source1/LConn1 -- threephase_vi_measures/LConn2
  Controlled Voltage Source2/LConn1 -- threephase_vi_measures/LConn3
  3ph_Dyg/LConn1 -- threephase_vi_measures/RConn1
  3ph_Dyg/LConn2 -- threephase_vi_measures/RConn2
  3ph_Dyg/LConn3 -- threephase_vi_measures/RConn3
  3ph_Dyg/RConn3 -- u3/RConn1
  3ph_Dyg/RConn2 -- u2/RConn1
  3ph_Dyg/RConn1 -- u1/RConn1

== system single_phase_inverter/grid/threephase_vi_measures ==
  Bus Creator : BusCreator  Inputs=6
  Bus Selector : BusSelector  OutputSignals=ia,ib,ic  OutputAsBus=on
  Bus Selector1 : BusSelector  OutputSignals=ua,ub,uc  OutputAsBus=on
  Current Sensor : fl_lib/Electrical/Electrical Sensors/Current Sensor
  Current Sensor1 : fl_lib/Electrical/Electrical Sensors/Current Sensor
  Current Sensor2 : fl_lib/Electrical/Electrical Sensors/Current Sensor
  Electrical Reference1 : fl_lib/Electrical/Electrical Elements/Electrical Reference
  Voltage Sensor : fl_lib/Electrical/Electrical Sensors/Voltage Sensor
  Voltage Sensor1 : fl_lib/Electrical/Electrical Sensors/Voltage Sensor
  Voltage Sensor2 : fl_lib/Electrical/Electrical Sensors/Voltage Sensor
  ia_grid : nesl_utility/PS-Simulink Converter  PhysicalDomain=network_engine_domain  SubClassName=ps_output  LeftPortType=input  RightPortType=output  PseudoPeriodic=off  Frequencies=[]  VectorFormat=1-D array  Unit=A  AffineConversion=off
  ib_grid : nesl_utility/PS-Simulink Converter  PhysicalDomain=network_engine_domain  SubClassName=ps_output  LeftPortType=input  RightPortType=output  PseudoPeriodic=off  Frequencies=[]  VectorFormat=1-D array  Unit=A  AffineConversion=off
  ic_grid : nesl_utility/PS-Simulink Converter  PhysicalDomain=network_engine_domain  SubClassName=ps_output  LeftPortType=input  RightPortType=output  PseudoPeriodic=off  Frequencies=[]  VectorFormat=1-D array  Unit=A  AffineConversion=off
  ua_grid : nesl_utility/PS-Simulink Converter  PhysicalDomain=network_engine_domain  SubClassName=ps_output  LeftPortType=input  RightPortType=output  PseudoPeriodic=off  Frequencies=[]  VectorFormat=1-D array  Unit=V  AffineConversion=off
  ub_grid : nesl_utility/PS-Simulink Converter  PhysicalDomain=network_engine_domain  SubClassName=ps_output  LeftPortType=input  RightPortType=output  PseudoPeriodic=off  Frequencies=[]  VectorFormat=1-D array  Unit=V  AffineConversion=off
  uc_grid : nesl_utility/PS-Simulink Converter  PhysicalDomain=network_engine_domain  SubClassName=ps_output  LeftPortType=input  RightPortType=output  PseudoPeriodic=off  Frequencies=[]  VectorFormat=1-D array  Unit=V  AffineConversion=off
  Ua : PMIOPort  Side=Left
  ua : PMIOPort  Port=2  Side=Right
  Ub : PMIOPort  Port=3  Side=Left
  ub : PMIOPort  Port=4  Side=Right
  Uc : PMIOPort  Port=5  Side=Left
  uc : PMIOPort  Port=6  Side=Right
  tag scope: ig_abc=global, ug_abc=global
  wires:
  Bus Selector1/1 -> [ug_abc]
  ib_grid/1 -> Bus Creator/5  "ib"
  ia_grid/1 -> Bus Creator/4  "ia"
  ic_grid/1 -> Bus Creator/6  "ic"
  ua_grid/1 -> Bus Creator/1  "ua"
  ub_grid/1 -> Bus Creator/2  "ub"
  uc_grid/1 -> Bus Creator/3  "uc"
  Bus Selector/1 -> [ig_abc]
  Bus Creator/1 -> Bus Selector/1, Bus Selector1/1  "vi_data"
  connections:
  Current Sensor1/LConn1 -- Ub/RConn1 -- Voltage Sensor1/LConn1
  Electrical Reference1/LConn1 -- Voltage Sensor/RConn2 -- Voltage Sensor2/RConn2 -- Voltage Sensor1/RConn2
  Voltage Sensor/RConn1 -- ua_grid/LConn1
  Current Sensor/RConn2 -- ua/RConn1
  Voltage Sensor1/RConn1 -- ub_grid/LConn1
  Voltage Sensor2/LConn1 -- Current Sensor2/LConn1 -- Uc/RConn1
  Current Sensor/LConn1 -- Ua/RConn1 -- Voltage Sensor/LConn1
  Current Sensor1/RConn2 -- ub/RConn1
  Voltage Sensor2/RConn1 -- uc_grid/LConn1
  ib_grid/LConn1 -- Current Sensor1/RConn1
  ia_grid/LConn1 -- Current Sensor/RConn1
  ic_grid/LConn1 -- Current Sensor2/RConn1
  Current Sensor2/RConn2 -- uc/RConn1

== system single_phase_inverter/rectifier/H5_filter ==
  Capacitor : fl_lib/Electrical/Electrical Elements/Capacitor  c=C5 F  r=1e-6 Ohm  g=0 1/Ohm  i_specify=off  i_priority=None  i=0 A  i_nominal_specify=off  i_nominal_value=1  i_nominal_unit=A  v_specify=off  v_priority=None  v=0 V  v_nominal_specify=off  v_nominal_value=1  v_nominal_unit=V  vc_specify=off  vc_priority=High  vc=0 V  vc_nominal_specify=off  vc_nominal_value=1  vc_nominal_unit=V
  Capacitor1 : fl_lib/Electrical/Electrical Elements/Capacitor  c=C5 F  r=1e-6 Ohm  g=0 1/Ohm  i_specify=off  i_priority=None  i=0 A  i_nominal_specify=off  i_nominal_value=1  i_nominal_unit=A  v_specify=off  v_priority=None  v=0 V  v_nominal_specify=off  v_nominal_value=1  v_nominal_unit=V  vc_specify=off  vc_priority=High  vc=0 V  vc_nominal_specify=off  vc_nominal_value=1  vc_nominal_unit=V
  Capacitor2 : fl_lib/Electrical/Electrical Elements/Capacitor  c=C5 F  r=1e-6 Ohm  g=0 1/Ohm  i_specify=off  i_priority=None  i=0 A  i_nominal_specify=off  i_nominal_value=1  i_nominal_unit=A  v_specify=off  v_priority=None  v=0 V  v_nominal_specify=off  v_nominal_value=1  v_nominal_unit=V  vc_specify=off  vc_priority=High  vc=0 V  vc_nominal_specify=off  vc_nominal_value=1  vc_nominal_unit=V
  Inductor5 : fl_lib/Electrical/Electrical Elements/Inductor  l=L5 H  r=0 Ohm  g=1e-9 1/Ohm  i_specify=off  i_priority=None  i=0 A  i_nominal_specify=off  i_nominal_value=1  i_nominal_unit=A  v_specify=off  v_priority=None  v=0 V  v_nominal_specify=off  v_nominal_value=1  v_nominal_unit=V  i_L_specify=off  i_L_priority=High  i_L=0 A  i_L_nominal_specify=off  i_L_nominal_value=1  i_L_nominal_unit=A
  Inductor6 : fl_lib/Electrical/Electrical Elements/Inductor  l=L5 H  r=0 Ohm  g=1e-9 1/Ohm  i_specify=off  i_priority=None  i=0 A  i_nominal_specify=off  i_nominal_value=1  i_nominal_unit=A  v_specify=off  v_priority=None  v=0 V  v_nominal_specify=off  v_nominal_value=1  v_nominal_unit=V  i_L_specify=off  i_L_priority=High  i_L=0 A  i_L_nominal_specify=off  i_L_nominal_value=1  i_L_nominal_unit=A
  Inductor7 : fl_lib/Electrical/Electrical Elements/Inductor  l=L5 H  r=0 Ohm  g=1e-9 1/Ohm  i_specify=off  i_priority=None  i=0 A  i_nominal_specify=off  i_nominal_value=1  i_nominal_unit=A  v_specify=off  v_priority=None  v=0 V  v_nominal_specify=off  v_nominal_value=1  v_nominal_unit=V  i_L_specify=off  i_L_priority=High  i_L=0 A  i_L_nominal_specify=off  i_L_nominal_value=1  i_L_nominal_unit=A
  w : PMIOPort  Side=Left
  v : PMIOPort  Port=2  Side=Left
  u : PMIOPort  Port=3  Side=Left
  connections:
  Capacitor2/LConn1 -- Inductor7/RConn1
  Inductor5/LConn1 -- w/RConn1
  Capacitor/RConn1 -- Capacitor2/RConn1 -- Capacitor1/RConn1
  Capacitor/LConn1 -- Inductor5/RConn1
  Capacitor1/LConn1 -- Inductor6/RConn1
  Inductor7/LConn1 -- u/RConn1
  Inductor6/LConn1 -- v/RConn1

== system single_phase_inverter/rectifier/H7_filter ==
  Capacitor1 : fl_lib/Electrical/Electrical Elements/Capacitor  c=C7 F  r=1e-6 Ohm  g=0 1/Ohm  i_specify=off  i_priority=None  i=0 A  i_nominal_specify=off  i_nominal_value=1  i_nominal_unit=A  v_specify=off  v_priority=None  v=0 V  v_nominal_specify=off  v_nominal_value=1  v_nominal_unit=V  vc_specify=off  vc_priority=High  vc=0 V  vc_nominal_specify=off  vc_nominal_value=1  vc_nominal_unit=V
  Capacitor2 : fl_lib/Electrical/Electrical Elements/Capacitor  c=C7 F  r=1e-6 Ohm  g=0 1/Ohm  i_specify=off  i_priority=None  i=0 A  i_nominal_specify=off  i_nominal_value=1  i_nominal_unit=A  v_specify=off  v_priority=None  v=0 V  v_nominal_specify=off  v_nominal_value=1  v_nominal_unit=V  vc_specify=off  vc_priority=High  vc=0 V  vc_nominal_specify=off  vc_nominal_value=1  vc_nominal_unit=V
  Capacitor3 : fl_lib/Electrical/Electrical Elements/Capacitor  c=C7 F  r=1e-6 Ohm  g=0 1/Ohm  i_specify=off  i_priority=None  i=0 A  i_nominal_specify=off  i_nominal_value=1  i_nominal_unit=A  v_specify=off  v_priority=None  v=0 V  v_nominal_specify=off  v_nominal_value=1  v_nominal_unit=V  vc_specify=off  vc_priority=High  vc=0 V  vc_nominal_specify=off  vc_nominal_value=1  vc_nominal_unit=V
  Inductor1 : fl_lib/Electrical/Electrical Elements/Inductor  l=L7 H  r=0 Ohm  g=1e-9 1/Ohm  i_specify=off  i_priority=None  i=0 A  i_nominal_specify=off  i_nominal_value=1  i_nominal_unit=A  v_specify=off  v_priority=None  v=0 V  v_nominal_specify=off  v_nominal_value=1  v_nominal_unit=V  i_L_specify=off  i_L_priority=High  i_L=0 A  i_L_nominal_specify=off  i_L_nominal_value=1  i_L_nominal_unit=A
  Inductor2 : fl_lib/Electrical/Electrical Elements/Inductor  l=L7 H  r=0 Ohm  g=1e-9 1/Ohm  i_specify=off  i_priority=None  i=0 A  i_nominal_specify=off  i_nominal_value=1  i_nominal_unit=A  v_specify=off  v_priority=None  v=0 V  v_nominal_specify=off  v_nominal_value=1  v_nominal_unit=V  i_L_specify=off  i_L_priority=High  i_L=0 A  i_L_nominal_specify=off  i_L_nominal_value=1  i_L_nominal_unit=A
  Inductor7 : fl_lib/Electrical/Electrical Elements/Inductor  l=L7 H  r=0 Ohm  g=1e-9 1/Ohm  i_specify=off  i_priority=None  i=0 A  i_nominal_specify=off  i_nominal_value=1  i_nominal_unit=A  v_specify=off  v_priority=None  v=0 V  v_nominal_specify=off  v_nominal_value=1  v_nominal_unit=V  i_L_specify=off  i_L_priority=High  i_L=0 A  i_L_nominal_specify=off  i_L_nominal_value=1  i_L_nominal_unit=A
  w : PMIOPort  Side=Left
  v : PMIOPort  Port=2  Side=Left
  u : PMIOPort  Port=3  Side=Left
  connections:
  Inductor1/LConn1 -- v/RConn1
  Inductor7/LConn1 -- u/RConn1
  Capacitor1/LConn1 -- Inductor1/RConn1
  Capacitor3/LConn1 -- Inductor2/RConn1
  Capacitor2/RConn1 -- Capacitor3/RConn1 -- Capacitor1/RConn1
  Inductor2/LConn1 -- w/RConn1
  Capacitor2/LConn1 -- Inductor7/RConn1

== system single_phase_inverter/single_phase_inverter/single phase inverter ==
  gate_commands : Inport
  Bus Selector : BusSelector  OutputSignals=mosfet_ploss_Q1,mosfet_voltage_Q1,mosfet_current_Q1,mosfet_JH_temp_Q1,mosfet_HA_temp_Q1
  Bus Selector1 : BusSelector  OutputSignals=mosfet_ploss_Q2,mosfet_voltage_Q2,mosfet_current_Q2,mosfet_JH_temp_Q2,mosfet_HA_temp_Q2
  full-bridge mosfet based with thermal model : full_bridge_mosfet_based_with_thermal_model/full-bridge mosfet based with thermal model  mass_heatsink_m=heatsink.no_weight  specific_heat_m=heatsink.cp  rth_mosfet_HA_m=heatsink.Rth_mosfet_HA  rth_mosfet_JH_m=mosfet.inv.Rth_mosfet_JH  Rds_on_m=mosfet.inv.Rds_on  Vth_m=mosfet.inv.Vth  Eon_m=mosfet.inv.Eon  Eoff_m=mosfet.inv.Eoff  Voff_sw_loss_m=mosfet.inv.Voff_sw_losses  Ion_sw_loss_m=mosfet.inv.Ion_sw_losses  Vdon_diode_m=mosfet.inv.Vdon_diode  Rdon_diode_m=mosfet.inv.Rdon_diode  JunctionTermalMass_m=mosfet.inv.JunctionTermalMass  Tambient_m=heatsink.Tambient  DThs_init_m=heatsink.DThs_init
  uac_out(+) : PMIOPort  Side=Left
  uac_out(-) : PMIOPort  Port=2  Side=Left
  udc(+) : PMIOPort  Port=3  Side=Right
  udc(-) : PMIOPort  Port=4  Side=Right
  tag scope: mosfet_HA_temp_invQ1=global, mosfet_HA_temp_invQ2=global, mosfet_JH_temp_invQ1=global, mosfet_JH_temp_invQ2=global, mosfet_current_invQ1=global, mosfet_current_invQ2=global, mosfet_ploss_invQ1=global, mosfet_ploss_invQ2=global, mosfet_voltage_invQ1=global, mosfet_voltage_invQ2=global
  wires:
  gate_commands/1 -> full-bridge mosfet based with thermal model/1
  Bus Selector/5 -> [mosfet_HA_temp_invQ1]  "<mosfet_HA_temp_Q1>"
  Bus Selector/4 -> [mosfet_JH_temp_invQ1]  "<mosfet_JH_temp_Q1>"
  Bus Selector/3 -> [mosfet_current_invQ1]  "<mosfet_current_Q1>"
  Bus Selector/2 -> [mosfet_voltage_invQ1]  "<mosfet_voltage_Q1>"
  Bus Selector/1 -> [mosfet_ploss_invQ1]  "<mosfet_ploss_Q1>"
  Bus Selector1/1 -> [mosfet_ploss_invQ2]  "<mosfet_ploss_Q2>"
  Bus Selector1/2 -> [mosfet_voltage_invQ2]  "<mosfet_voltage_Q2>"
  Bus Selector1/3 -> [mosfet_current_invQ2]  "<mosfet_current_Q2>"
  Bus Selector1/4 -> [mosfet_JH_temp_invQ2]  "<mosfet_JH_temp_Q2>"
  Bus Selector1/5 -> [mosfet_HA_temp_invQ2]  "<mosfet_HA_temp_Q2>"
  full-bridge mosfet based with thermal model/1 -> Bus Selector1/1, Bus Selector/1
  connections:
  full-bridge mosfet based with thermal model/RConn2 -- uac_out(-)/RConn1
  full-bridge mosfet based with thermal model/LConn1 -- udc(+)/RConn1
  full-bridge mosfet based with thermal model/RConn1 -- uac_out(+)/RConn1
  full-bridge mosfet based with thermal model/LConn2 -- udc(-)/RConn1

== system single_phase_inverter/single_phase_inverter/single phase inverter control ==
  acquisition_and_scaling_current : Subsystem  Commented=on
  acquisition_and_scaling_current_with_white_noise : Subsystem
  acquisition_and_scaling_dc_voltage : Subsystem
  acquisition_and_scaling_grid_voltage_ac : Subsystem
  acquisition_and_scaling_voltage : Subsystem
  inverter_current_output_pu_reference : Subsystem
  pwm modulator : Subsystem
  single_phase_inverter_ctrl : Subsystem
  gate_cmds : Outport
  wires:
  [inverter_current_output] -> acquisition_and_scaling_current_with_white_noise/1(in)
  pwm modulator/1(gate_cmds) -> gate_cmds/1
  [TRGO_INV_1] -> single_phase_inverter_ctrl/Trigger
  [inverter_voltage_output] -> acquisition_and_scaling_voltage/1(in)
  single_phase_inverter_ctrl/1(u_ctrl_out) -> pwm modulator/1(vout)
  acquisition_and_scaling_current_with_white_noise/1(out) -> single_phase_inverter_ctrl/2(inverter_current_output_pu)  "inverter_current_output_pu"
  acquisition_and_scaling_voltage/1(out) -> single_phase_inverter_ctrl/1(inverter_voltage_output_pu)  "inverter_voltage_output_pu"
  inverter_current_output_pu_reference/1(inverter_current_output_pu_reference) -> single_phase_inverter_ctrl/3(inverter_current output_pu_reference)  "inverter_current_output_pu_reference"
  [dclink_voltage] -> acquisition_and_scaling_dc_voltage/1(in)
  acquisition_and_scaling_dc_voltage/1(out) -> single_phase_inverter_ctrl/4(dclink_voltage_pu)  "dclink_voltage_pu"
  [time_inv_module_1] -> single_phase_inverter_ctrl/5(local_time)
  [ug_abc] -> acquisition_and_scaling_grid_voltage_ac/1(in)
  acquisition_and_scaling_grid_voltage_ac/1(out) -> single_phase_inverter_ctrl/6(ugrid_pu)  "ug_abc"
